simulink model "furuta_rl_training"  (R2026b)
settings: Solver=FixedStepDiscrete  StopTime=5  FixedStep=controlPeriod
model workspace (MAT data in the model file):
  agentKind = "PPO (초기 정책)"
  controlPeriod = 0.01
  controllerMode = 1
  furutaAgent : rl.agent.rlPPOAgent (value not decoded)
  furutaToolboxMpc = mpc
  furutaToolboxMpc.Ts = 0.01
  furutaToolboxMpc.PredictionHorizon = 20
  furutaToolboxMpc.ControlHorizon = 20
  furutaToolboxMpc.Model.Plant = ss
  furutaToolboxMpc.Model.Plant.InputName_ = "MV1"
  furutaToolboxMpc.Model.Plant.InputGroup_.Manipulated = 1
  furutaToolboxMpc.Model.Plant.OutputName_ = ["MO1"; "MO2"; "MO3"; "MO4"; "MO5"; "MO6"; "MO7"; "MO8"]
  furutaToolboxMpc.Model.Plant.OutputGroup_.Measured = [1 2 3 4 5 6 7 8]
  furutaToolboxMpc.Model.Plant.IOSize_ = [8 1]
  furutaToolboxMpc.Model.Plant.Data_ = ltipack.ssdata
  furutaToolboxMpc.Model.Plant.Data_.a = [1  -0.00902674267589  0.00993774320897  -2.4767657698e-05; 0  1.0129802947  5.33054368483e-05  0.0100355972733; 0  -1.80504476453  0.987560350231  -0.00796081332398; 0  2.59780112786  0.0106592935191  1.01144622057]
  furutaToolboxMpc.Model.Plant.Data_.c = [1  0  0  0; 0  1  0  0; 0  0  1  0; 0  0  0  1; 23.187012799  50.483540443  3.96076595787  4.74600329341; 0  69.1342012244  4.52520194197  5.64653884547; 0  0  1.92549619263  1.610475723; 0  0  0  1.43133536407]
  furutaToolboxMpc.Model.Plant.Data_.dx0 = [0; 0; 0; 0]
  furutaToolboxMpc.Model.Plant.Data_.x0 = [0; 0; 0; 0]
  furutaToolboxMpc.Model.Plant.Data_.b = [0.0186770373086; -0.0159916310545; 3.73189493068; -3.19778805573]
  furutaToolboxMpc.Model.Plant.Data_.d = [0; 0; 0; 0; 0; 0; 0; 0]
  furutaToolboxMpc.Model.Plant.Data_.u0 = 0
  furutaToolboxMpc.Model.Plant.Data_.y0 = [0; 0; 0; 0; 0; 0; 0; 0]
  furutaToolboxMpc.Model.Plant.Data_.Delay.Input = 0
  furutaToolboxMpc.Model.Plant.Data_.Delay.Output = [0; 0; 0; 0; 0; 0; 0; 0]
  furutaToolboxMpc.Model.Plant.Data_.Delay.Internal = []
  furutaToolboxMpc.Model.Plant.Data_.Ts = 0.01
  furutaToolboxMpc.Model.Disturbance = []
  furutaToolboxMpc.Model.Noise = []
  furutaToolboxMpc.Model.Nominal.X = [0; 0; 0; 0]
  furutaToolboxMpc.Model.Nominal.DX = [0; 0; 0; 0]
  furutaToolboxMpc.Model.Nominal.U = 0
  furutaToolboxMpc.Model.Nominal.Y = [0; 0; 0; 0; 0; 0; 0; 0]
  furutaToolboxMpc.ManipulatedVariables.Min = [-1; -1; -1; -1; -1; -1; -1; -1; -1; -1; -1; -1; -1; -1; -1; -1; -1; -1; -1; -1]
  furutaToolboxMpc.ManipulatedVariables.Max = [1; 1; 1; 1; 1; 1; 1; 1; 1; 1; 1; 1; 1; 1; 1; 1; 1; 1; 1; 1]
  furutaToolboxMpc.ManipulatedVariables.MinECR = [0; 0; 0; 0; 0; 0; 0; 0; 0; 0; 0; 0; 0; 0; 0; 0; 0; 0; 0; 0]
  furutaToolboxMpc.ManipulatedVariables.MaxECR = [0; 0; 0; 0; 0; 0; 0; 0; 0; 0; 0; 0; 0; 0; 0; 0; 0; 0; 0; 0]
  furutaToolboxMpc.ManipulatedVariables.RateMin = -Inf
  furutaToolboxMpc.ManipulatedVariables.RateMax = Inf
  furutaToolboxMpc.ManipulatedVariables.RateMinECR = 0
  furutaToolboxMpc.ManipulatedVariables.RateMaxECR = 0
  furutaToolboxMpc.ManipulatedVariables.Target = 'nominal'
  furutaToolboxMpc.ManipulatedVariables.Name = 'MV1'
  furutaToolboxMpc.ManipulatedVariables.Units = ''
  furutaToolboxMpc.ManipulatedVariables.ScaleFactor = 1
  furutaToolboxMpc.ManipulatedVariables.Type = 'continuous'
  furutaToolboxMpc.OutputVariables(1).Min = [-Inf; -Inf; -Inf; -Inf; -Inf; -Inf; -Inf; -Inf; -Inf; -Inf; -Inf; -Inf; -Inf; -Inf; -Inf; -Inf; -Inf; -Inf; -Inf; -Inf]
  furutaToolboxMpc.OutputVariables(1).Max = [Inf; Inf; Inf; Inf; Inf; Inf; Inf; Inf; Inf; Inf; Inf; Inf; Inf; Inf; Inf; Inf; Inf; Inf; Inf; Inf]
  furutaToolboxMpc.OutputVariables(1).MinECR = [2; 2; 2; 2; 2; 2; 2; 2; 2; 2; 2; 2; 2; 2; 2; 2; 2; 2; 2; 2]
  furutaToolboxMpc.OutputVariables(1).MaxECR = [2; 2; 2; 2; 2; 2; 2; 2; 2; 2; 2; 2; 2; 2; 2; 2; 2; 2; 2; 2]
  furutaToolboxMpc.OutputVariables(1).Name = 'MO1'
  furutaToolboxMpc.OutputVariables(1).Units = ''
  furutaToolboxMpc.OutputVariables(1).ScaleFactor = 1
  furutaToolboxMpc.OutputVariables(2).Min = [-Inf; -Inf; -Inf; -Inf; -Inf; -Inf; -Inf; -Inf; -Inf; -Inf; -Inf; -Inf; -Inf; -Inf; -Inf; -Inf; -Inf; -Inf; -Inf; -Inf]
  furutaToolboxMpc.OutputVariables(2).Max = [Inf; Inf; Inf; Inf; Inf; Inf; Inf; Inf; Inf; Inf; Inf; Inf; Inf; Inf; Inf; Inf; Inf; Inf; Inf; Inf]
  furutaToolboxMpc.OutputVariables(2).MinECR = [2; 2; 2; 2; 2; 2; 2; 2; 2; 2; 2; 2; 2; 2; 2; 2; 2; 2; 2; 2]
  furutaToolboxMpc.OutputVariables(2).MaxECR = [2; 2; 2; 2; 2; 2; 2; 2; 2; 2; 2; 2; 2; 2; 2; 2; 2; 2; 2; 2]
  furutaToolboxMpc.OutputVariables(2).Name = 'MO2'
  furutaToolboxMpc.OutputVariables(2).Units = ''
  furutaToolboxMpc.OutputVariables(2).ScaleFactor = 1
  furutaToolboxMpc.OutputVariables(3).Min = [-Inf; -Inf; -Inf; -Inf; -Inf; -Inf; -Inf; -Inf; -Inf; -Inf; -Inf; -Inf; -Inf; -Inf; -Inf; -Inf; -Inf; -Inf; -Inf; -Inf]
  furutaToolboxMpc.OutputVariables(3).Max = [Inf; Inf; Inf; Inf; Inf; Inf; Inf; Inf; Inf; Inf; Inf; Inf; Inf; Inf; Inf; Inf; Inf; Inf; Inf; Inf]
  furutaToolboxMpc.OutputVariables(3).MinECR = [2; 2; 2; 2; 2; 2; 2; 2; 2; 2; 2; 2; 2; 2; 2; 2; 2; 2; 2; 2]
  furutaToolboxMpc.OutputVariables(3).MaxECR = [2; 2; 2; 2; 2; 2; 2; 2; 2; 2; 2; 2; 2; 2; 2; 2; 2; 2; 2; 2]
  furutaToolboxMpc.OutputVariables(3).Name = 'MO3'
  furutaToolboxMpc.OutputVariables(3).Units = ''
  furutaToolboxMpc.OutputVariables(3).ScaleFactor = 1
  furutaToolboxMpc.OutputVariables(4).Min = [-Inf; -Inf; -Inf; -Inf; -Inf; -Inf; -Inf; -Inf; -Inf; -Inf; -Inf; -Inf; -Inf; -Inf; -Inf; -Inf; -Inf; -Inf; -Inf; -Inf]
  furutaToolboxMpc.OutputVariables(4).Max = [Inf; Inf; Inf; Inf; Inf; Inf; Inf; Inf; Inf; Inf; Inf; Inf; Inf; Inf; Inf; Inf; Inf; Inf; Inf; Inf]
  furutaToolboxMpc.OutputVariables(4).MinECR = [2; 2; 2; 2; 2; 2; 2; 2; 2; 2; 2; 2; 2; 2; 2; 2; 2; 2; 2; 2]
  furutaToolboxMpc.OutputVariables(4).MaxECR = [2; 2; 2; 2; 2; 2; 2; 2; 2; 2; 2; 2; 2; 2; 2; 2; 2; 2; 2; 2]
  furutaToolboxMpc.OutputVariables(4).Name = 'MO4'
  furutaToolboxMpc.OutputVariables(4).Units = ''
  furutaToolboxMpc.OutputVariables(4).ScaleFactor = 1
  furutaToolboxMpc.OutputVariables(5).Min = [-Inf; -Inf; -Inf; -Inf; -Inf; -Inf; -Inf; -Inf; -Inf; -Inf; -Inf; -Inf; -Inf; -Inf; -Inf; -Inf; -Inf; -Inf; -Inf; -Inf]
  furutaToolboxMpc.OutputVariables(5).Max = [Inf; Inf; Inf; Inf; Inf; Inf; Inf; Inf; Inf; Inf; Inf; Inf; Inf; Inf; Inf; Inf; Inf; Inf; Inf; Inf]
  furutaToolboxMpc.OutputVariables(5).MinECR = [2; 2; 2; 2; 2; 2; 2; 2; 2; 2; 2; 2; 2; 2; 2; 2; 2; 2; 2; 2]
  furutaToolboxMpc.OutputVariables(5).MaxECR = [2; 2; 2; 2; 2; 2; 2; 2; 2; 2; 2; 2; 2; 2; 2; 2; 2; 2; 2; 2]
  furutaToolboxMpc.OutputVariables(5).Name = 'MO5'
  furutaToolboxMpc.OutputVariables(5).Units = ''
  furutaToolboxMpc.OutputVariables(5).ScaleFactor = 1
  furutaToolboxMpc.OutputVariables(6).Min = [-Inf; -Inf; -Inf; -Inf; -Inf; -Inf; -Inf; -Inf; -Inf; -Inf; -Inf; -Inf; -Inf; -Inf; -Inf; -Inf; -Inf; -Inf; -Inf; -Inf]
  furutaToolboxMpc.OutputVariables(6).Max = [Inf; Inf; Inf; Inf; Inf; Inf; Inf; Inf; Inf; Inf; Inf; Inf; Inf; Inf; Inf; Inf; Inf; Inf; Inf; Inf]
  furutaToolboxMpc.OutputVariables(6).MinECR = [2; 2; 2; 2; 2; 2; 2; 2; 2; 2; 2; 2; 2; 2; 2; 2; 2; 2; 2; 2]
  furutaToolboxMpc.OutputVariables(6).MaxECR = [2; 2; 2; 2; 2; 2; 2; 2; 2; 2; 2; 2; 2; 2; 2; 2; 2; 2; 2; 2]
  furutaToolboxMpc.OutputVariables(6).Name = 'MO6'
  furutaToolboxMpc.OutputVariables(6).Units = ''
  furutaToolboxMpc.OutputVariables(6).ScaleFactor = 1
  furutaToolboxMpc.OutputVariables(7).Min = [-Inf; -Inf; -Inf; -Inf; -Inf; -Inf; -Inf; -Inf; -Inf; -Inf; -Inf; -Inf; -Inf; -Inf; -Inf; -Inf; -Inf; -Inf; -Inf; -Inf]
  furutaToolboxMpc.OutputVariables(7).Max = [Inf; Inf; Inf; Inf; Inf; Inf; Inf; Inf; Inf; Inf; Inf; Inf; Inf; Inf; Inf; Inf; Inf; Inf; Inf; Inf]
  furutaToolboxMpc.OutputVariables(7).MinECR = [2; 2; 2; 2; 2; 2; 2; 2; 2; 2; 2; 2; 2; 2; 2; 2; 2; 2; 2; 2]
  furutaToolboxMpc.OutputVariables(7).MaxECR = [2; 2; 2; 2; 2; 2; 2; 2; 2; 2; 2; 2; 2; 2; 2; 2; 2; 2; 2; 2]
  furutaToolboxMpc.OutputVariables(7).Name = 'MO7'
  furutaToolboxMpc.OutputVariables(7).Units = ''
  furutaToolboxMpc.OutputVariables(7).ScaleFactor = 1
  furutaToolboxMpc.OutputVariables(8).Min = [-Inf; -Inf; -Inf; -Inf; -Inf; -Inf; -Inf; -Inf; -Inf; -Inf; -Inf; -Inf; -Inf; -Inf; -Inf; -Inf; -Inf; -Inf; -Inf; -Inf]
  furutaToolboxMpc.OutputVariables(8).Max = [Inf; Inf; Inf; Inf; Inf; Inf; Inf; Inf; Inf; Inf; Inf; Inf; Inf; Inf; Inf; Inf; Inf; Inf; Inf; Inf]
  furutaToolboxMpc.OutputVariables(8).MinECR = [2; 2; 2; 2; 2; 2; 2; 2; 2; 2; 2; 2; 2; 2; 2; 2; 2; 2; 2; 2]
  furutaToolboxMpc.OutputVariables(8).MaxECR = [2; 2; 2; 2; 2; 2; 2; 2; 2; 2; 2; 2; 2; 2; 2; 2; 2; 2; 2; 2]
  furutaToolboxMpc.OutputVariables(8).Name = 'MO8'
  furutaToolboxMpc.OutputVariables(8).Units = ''
  furutaToolboxMpc.OutputVariables(8).ScaleFactor = 1
  furutaToolboxMpc.Weights.ManipulatedVariables = [1; 1; 1; 1; 1; 1; 1; 1; 1; 1; 1; 1; 1; 1; 1; 1; 1; 1; 1; 1]
  furutaToolboxMpc.Weights.ManipulatedVariablesRate = 1e-05
  furutaToolboxMpc.Weights.OutputVariables = [3.16227766017  3.16227766017  1  1  0  0  0  0; 3.16227766017  3.16227766017  1  1  0  0  0  0; 3.16227766017  3.16227766017  1  1  0  0  0  0; 3.16227766017  3.16227766017  1  1  0  0  0  0; 3.16227766017  3.16227766017  1  1  0  0  0  0; 3.16227766017  3.16227766017  1  1  0  0  0  0; 3.16227766017  3.16227766017  1  1  0  0  0  0; 3.16227766017  3.16227766017  1  1  0  0  0  0; 3.16227766017  3.16227766017  1  1  0  0  0  0; 3.16227766017  3.16227766017  1  1  0  0  0  0; 3.16227766017  3.16227766017  1  1  0  0  0  0; 3.16227766017  3.16227766017  1  1  0  0  0  0; 3.16227766017  3.16227766017  1  1  0  0  0  0; 3.16227766017  3.16227766017  1  1  0  0  0  0; 3.16227766017  3.16227766017  1  1  0  0  0  0; 3.16227766017  3.16227766017  1  1  0  0  0  0; 3.16227766017  3.16227766017  1  1  0  0  0  0; 3.16227766017  3.16227766017  1  1  0  0  0  0; 3.16227766017  3.16227766017  1  1  0  0  0  0; 0  0  0  0  1  1  1  1]
  furutaToolboxMpc.Weights.ECR = 100000
  furutaToolboxMpc.Optimizer.OptimizationType = 'QP'
  furutaToolboxMpc.Optimizer.Solver = 'active-set'
  furutaToolboxMpc.Optimizer.SolverOptions = mpc.solver.options.qp.ActiveSet
  furutaToolboxMpc.Optimizer.SolverOptions.SolverName = 'ActiveSet'
  furutaToolboxMpc.Optimizer.MinOutputECR = 0
  furutaToolboxMpc.Optimizer.UseSuboptimalSolution = 0
  furutaToolboxMpc.Optimizer.CustomSolver = 0
  furutaToolboxMpc.Optimizer.CustomSolverCodeGen = 0
  furutaToolboxMpc.History = [2026 11 18 15 19 42.726]
  furutaToolboxMpc.MPCData = mpcdata
  furutaToolboxMpc.MPCData.IsDirty = 1
  furutaToolboxMpc.MPCData.Ts = 0.01
  furutaToolboxMpc.MPCData.p = 20
  furutaToolboxMpc.MPCData.m = 20
  furutaToolboxMpc.MPCData.UseActiveSetSolver = 1
  furutaToolboxMpc.MPCData.UseSuboptimalSolution = 0
  furutaToolboxMpc.MPCData.CustomSolver = 0
  furutaToolboxMpc.MPCData.CustomSolverCodeGen = 0
  furutaToolboxMpc.MPCData.IsCustomEstimation = 1
  furutaToolboxMpc.MPCData.Uscale = 1
  furutaToolboxMpc.MPCData.Yscale = [1; 1; 1; 1; 1; 1; 1; 1]
  furutaToolboxMpc.MPCData.mvindex = 1
  furutaToolboxMpc.MPCData.myindex = [1; 2; 3; 4; 5; 6; 7; 8]
  furutaToolboxMpc.MPCData.ASOptions.MaxIterations = 120
  furutaToolboxMpc.MPCData.ASOptions.MaxTime = Inf
  furutaToolboxMpc.MPCData.ASOptions.ConstraintTolerance = 1e-06
  furutaToolboxMpc.MPCData.ASOptions.UseWarmStart = 1
  furutaToolboxMpc.MPCData.IPOptions.MaxIterations = 50
  furutaToolboxMpc.MPCData.IPOptions.MaxTime = Inf
  furutaToolboxMpc.MPCData.IPOptions.ConstraintTolerance = 1e-06
  furutaToolboxMpc.MPCData.IPOptions.OptimalityTolerance = 1e-06
  furutaToolboxMpc.MPCData.IPOptions.ComplementarityTolerance = 1e-08
  furutaToolboxMpc.MPCData.IPOptions.StepTolerance = 1e-08
  furutaToolboxMpc.MPCData.ADOptions.AbsoluteTolerance = 0.001
  furutaToolboxMpc.MPCData.ADOptions.RelativeTolerance = 0.001
  furutaToolboxMpc.MPCData.ADOptions.MaxIterations = 1000
  furutaToolboxMpc.MPCData.ADOptions.MaxTime = Inf
  furutaToolboxMpc.MPCData.ADOptions.RelaxationParameter = 1.6
  furutaToolboxMpc.MPCData.ADOptions.PenaltyParameter = 0.1
  furutaToolboxMpc.MPCData.ADOptions.StepSize = 1e-06
  furutaToolboxMpc.MPCData.ADOptions.PrimalInfeasibilityTolerance = 0.0001
  furutaToolboxMpc.MPCData.ADOptions.DualInfeasibilityTolerance = 0.0001
  furutaToolboxMpc.MPCData.ADOptions.EnablePolish = 0
  furutaToolboxMpc.MPCData.ADOptions.PolishRegularization = 1e-06
  furutaToolboxMpc.MPCData.ADOptions.PolishTolerance = 1e-08
  furutaToolboxMpc.MPCData.ADOptions.PolishMaxIterations = 3
  furutaToolboxMpc.MPCData.MIQPOptions.MaxIterations = 1000
  furutaToolboxMpc.MPCData.MIQPOptions.MaxTime = Inf
  furutaToolboxMpc.MPCData.MIQPOptions.ConstraintTolerance = 1e-06
  furutaToolboxMpc.MPCData.MIQPOptions.UseWarmStart = 0
  furutaToolboxMpc.MPCData.MIQPOptions.DiscreteConstraintTolerance = 1e-06
  furutaToolboxMpc.MPCData.MIQPOptions.RoundingAtRootNode = 1
  furutaToolboxMpc.MPCData.MIQPOptions.MaxPendingNodes = 1000
  furutaToolboxMpc.IsEmpty = 0
  furutaToolboxMpc.OldOVIntegrator = {[]; []; []; []; []; []; []; []}
  furutaToolboxMpc.EstGain = 'custom'
  furutaToolboxMpc.OutDistModel = ss
  furutaToolboxMpc.OutDistModel.IOSize_ = [8 1]
  furutaToolboxMpc.OutDistModel.Data_ = ltipack.ssdata
  furutaToolboxMpc.OutDistModel.Data_.d = [0; 0; 0; 0; 0; 0; 0; 0]
  furutaToolboxMpc.OutDistModel.Data_.u0 = 0
  furutaToolboxMpc.OutDistModel.Data_.y0 = [0; 0; 0; 0; 0; 0; 0; 0]
  furutaToolboxMpc.OutDistModel.Data_.Delay.Input = 0
  furutaToolboxMpc.OutDistModel.Data_.Delay.Output = [0; 0; 0; 0; 0; 0; 0; 0]
  furutaToolboxMpc.OutDistModel.Data_.Delay.Internal = []
  furutaToolboxMpc.OutDistModel.Data_.Ts = 0
  furutaToolboxMpc.Version = '26.2'
  initialState = [0; 0.174532925199; 0; 0]
  integrationStep = 0.002
  lmpcF = [-2830.68997815  -425545.566766  -3378.75183897  -27996.6485902; -2386.43056313  -361642.554145  -2861.88762577  -23784.8995788; -2007.92623528  -307039.935727  -2420.70891761  -20186.6799153; -1685.61022299  -260385.70884  -2044.21747245  -17112.76233; -1411.30389107  -220523.512325  -1723.00852583  -14486.8389364; -1178.01505811  -186464.084025  -1449.03879544  -12243.6357575; -979.765570681  -157360.828718  -1215.42801756  -10327.2990171; -811.443882151  -132488.892998  -1016.2891174  -8690.01329063; -668.67900017  -111227.229747  -846.5828196  -7290.81731336; -547.732694122  -93043.2082769  -701.993107015  -6094.58810591; -445.407303829  -77479.3885256  -578.820447971  -5071.16820406; -358.966875555  -64142.130684  -473.890148738  -4194.61428813; -286.069679883  -52691.7563221  -384.473558738  -3442.54847023; -224.710446621  -42834.0147656  -308.220170492  -2795.59599508; -173.170891379  -34312.6399545  -243.098922081  -2236.8951992; -129.97731279  -26902.8090841  -187.34723347  -1751.66730548; -93.8642135106  -20405.3356068  -139.426494783  -1326.83504718; -63.7430465086  -14641.4461488  -97.9828790679  -950.680248883; -38.6753142339  -9448.00396528  -61.8124779305  -612.531370742; -17.8493553576  -4673.05100156  -29.8298585475  -302.472662498]
  lmpcH = [71196.7632757 60515.4631775 51389.63963 43592.1776843 36929.7000861 31236.7872342 26371.8858267 22213.8049684 18658.7129743 15617.560407 13013.8653496 10781.8057824 ... (400 elements, 20x20)]
  lqrGain = [-0.560244322113 -7.30813603654 -0.304541725168 -0.68699829167]
  maxTorque = 0.03
  pidGains = [8.3479 0.5085 0.5811 0.3312 0.0475]
  plantCoefficients = [0.00019818 0.00016078 0.00016134 0.00013805 0.016934 0.0001 1e-05 0]
  poleGain = [-1.34079378819 -10.2715412157 -0.553426126336 -0.956316780761]
  rlRewardLevel = 2
  rmd.model = 'RMD-X6-P20-60-E'
  rmd.voltage = 48
  rmd.gearRatio = 19.612
  rmd.ratedTorque = 20
  rmd.ratedCurrent = 9.5
  rmd.ratedSpeedRPM = 153
  rmd.noLoadSpeedRPM = 176
  rmd.Kt = 2.1
  rmd.currentLSB = 0.01
  rmdCommandDelaySamples = 1
  rmdCurrentTimeConstant = 0
  scenarioStimulus = [0 0.0075 0.0175 0.0275 0.0375 0.0475 0.0575 0.0675 0.0775 0.0875 0.0975 0.1075 ... (2004 elements, 501x4)]
  usePolicyCallback = 0
  useRmd = 1
undefined symbols (not defined in the file or in its folder): sgn
libraries: mpclib x1, rllib x1
(part 1 of 2)
settings Model: Creator=Lsh  LastModifiedBy=Lsh

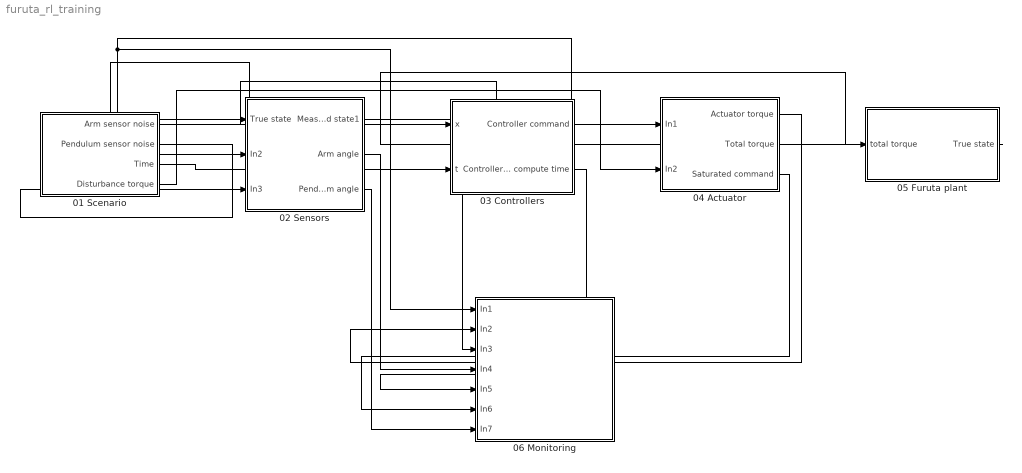
== system furuta_rl_training ==
  01 Scenario : Subsystem
  02 Sensors : Subsystem
  03 Controllers : Subsystem
  04 Actuator : Subsystem
  05 Furuta plant : Subsystem
  06 Monitoring : Subsystem
  wires:
  01 Scenario/1(Arm sensor noise) -> 02 Sensors/2(In2)
  01 Scenario/2(Pendulum sensor noise) -> 02 Sensors/3(In3)
  03 Controllers/1(Controller command) -> 06 Monitoring/3(In3), 04 Actuator/1(In1)
  02 Sensors/1(Measured state1) -> 03 Controllers/1(x)
  01 Scenario/3(Time) -> 03 Controllers/2(t)
  01 Scenario/4(Disturbance torque) -> 04 Actuator/2(In2)
  05 Furuta plant/1(True state) -> 06 Monitoring/1(In1), 02 Sensors/1(True state)
  04 Actuator/2(Total torque) -> 05 Furuta plant/1(total torque)
  04 Actuator/1(Actuator torque) -> 06 Monitoring/2(In2)
  02 Sensors/2(Arm angle) -> 06 Monitoring/4(In4)
  03 Controllers/2(Controller compute time) -> 06 Monitoring/5(In5)
  04 Actuator/3(Saturated command) -> 06 Monitoring/6(In6)
  02 Sensors/3(Pendulum angle) -> 06 Monitoring/7(In7)

== system furuta_rl_training/01 Scenario ==
  Clock : DigitalClock  SampleTime=controlPeriod
  Scenario : FromWorkspace  VariableName=scenarioStimulus  SampleTime=controlPeriod  Interpolate=off  OutputAfterFinalValue=Holding final value
  Scenario channels : Demux  Outputs=3
  Arm sensor noise : Outport
  Pendulum sensor noise : Outport  Port=2
  Time : Outport  Port=3
  Disturbance torque : Outport  Port=4
  wires:
  Scenario channels/1 -> Arm sensor noise/1  "Arm sensor noise"
  Clock/1 -> Time/1  "Time"
  Scenario/1 -> Scenario channels/1
  Scenario channels/3 -> Disturbance torque/1  "Disturbance torque"
  Scenario channels/2 -> Pendulum sensor noise/1  "Pendulum sensor noise"

== system furuta_rl_training/02 Sensors ==
  True state : Inport
  In2 : Inport  Port=2
  In3 : Inport  Port=3
  Measured arm : Sum
  Measured pendulum : Sum
  Measured state : Mux
  State channels : Demux
  Measured state1 : Outport
  Arm angle : Outport  Port=2
  Pendulum angle : Outport  Port=3
  wires:
  True state/1 -> State channels/1
  State channels/1 -> Arm angle/1, Measured arm/1  "Arm angle"
  Measured state/1 -> Measured state1/1  "Measured state"
  State channels/2 -> Pendulum angle/1, Measured pendulum/1  "Pendulum angle"
  Measured arm/1 -> Measured state/1
  Measured pendulum/1 -> Measured state/2
  State channels/4 -> Measured state/4
  State channels/3 -> Measured state/3
  In2/1 -> Measured arm/2
  In3/1 -> Measured pendulum/2

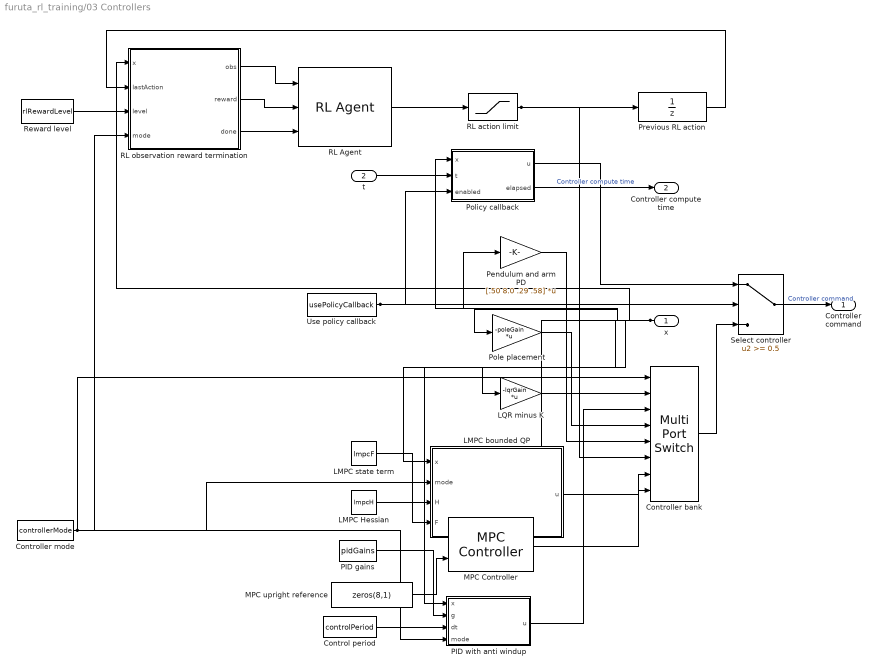
== system furuta_rl_training/03 Controllers ==
  x : Inport
  t : Inport  Port=2
  Control period : Constant  Value=controlPeriod
  Controller bank : MultiPortSwitch  Inputs=7  SaturateOnIntegerOverflow=off  InputSameDT=off
  Controller mode : Constant  Value=controllerMode
  LMPC Hessian : Constant  Value=lmpcH
  LMPC bounded QP : MATLAB Function  TreatAsAtomicUnit=on
  LMPC state term : Constant  Value=lmpcF
  LQR minus K : Gain  Gain=-lqrGain  Multiplication=Matrix(K*u) (u vector)
  MPC Controller : mpclib/MPC Controller  SCDEnableBlockLinearizationSpecification=on  mpcobj=furutaToolboxMpc  is_multiple=0  enable_value=0  return_u0=off  updateMPCinCallerWorkspace=on  md_inport=off  mv_inport=off  uref_inport=off  return_cost=off  return_mvseq=off  return_qpstatus=off  return_xseq=off  return_state=off  return_ovseq=off  state_inport=on  umin_inport=off  umax_inport=off  ymin_inport=off  ymax_inport=off  cc_inport=off  ywt_inport=off  uwt_inport=off  duwt_inport=off  rhoeps_inport=off  pm_inport=off  MaximumP=10  HorizonChoice=FixedHorizon  n_ts=1  n_p=10  n_mv=1  n_md=1  n_ud=0  n_mo=1  n_uo=0  BlockDataType=double  SampleTimeInherited=off  switch_inport=off
  MPC upright reference : Constant  Value=zeros(8,1)
  PID gains : Constant  Value=pidGains
  PID with anti windup : MATLAB Function  TreatAsAtomicUnit=on
  Pendulum and arm PD : Gain  Gain=[.50 8.0 .29 .58]  Multiplication=Matrix(K*u) (u vector)
  Pole placement : Gain  Gain=-poleGain  Multiplication=Matrix(K*u) (u vector)
  Policy callback : MATLAB Function  TreatAsAtomicUnit=on
  Previous RL action : UnitDelay  SampleTime=controlPeriod
  RL Agent : rllib/RL Agent  Agent=furutaAgent  ExternalActionAsInput=off  ProvideLastAction=off  ProvideCumRwd=off  TreatAsDirectFeedthrough=on  UseStrictObservationDataTypes=off
  RL action limit : Saturate  UpperLimit=1  LowerLimit=-1
  RL observation reward termination : MATLAB Function  TreatAsAtomicUnit=on
  Reward level : Constant  Value=rlRewardLevel
  Select controller : Switch  Threshold=0.5  SaturateOnIntegerOverflow=off  InputSameDT=off
  Use policy callback : Constant  Value=usePolicyCallback
  Controller command : Outport
  Controller compute time : Outport  Port=2
  wires:
  Reward level/1 -> RL observation reward termination/3(level)
  RL observation reward termination/2(reward) -> RL Agent/2
  Controller mode/1 -> PID with anti windup/4(mode), LMPC bounded QP/2(mode), Controller bank/1, RL observation reward termination/4(mode)
  LMPC Hessian/1 -> LMPC bounded QP/3(H)
  Use policy callback/1 -> Select controller/2, Policy callback/3(enabled)
  RL observation reward termination/1(obs) -> RL Agent/1
  RL observation reward termination/3(done) -> RL Agent/3
  RL Agent/1 -> RL action limit/1
  t/1 -> Policy callback/2(t)
  LMPC state term/1 -> LMPC bounded QP/4(F)
  PID gains/1 -> PID with anti windup/2(g)
  Control period/1 -> PID with anti windup/3(dt)
  RL action limit/1 -> Previous RL action/1, Controller bank/6
  Policy callback/1(u) -> Select controller/1
  Policy callback/2(elapsed) -> Controller compute time/1  "Controller compute time"
  Pendulum and arm PD/1 -> Controller bank/5
  Pole placement/1 -> Controller bank/4
  LQR minus K/1 -> Controller bank/2
  LMPC bounded QP/1(u) -> Controller bank/7
  Select controller/1 -> Controller command/1  "Controller command"
  PID with anti windup/1(u) -> Controller bank/3
  x/1 -> Pole placement/1, LQR minus K/1, LMPC bounded QP/1(x), Policy callback/1(x), Pendulum and arm PD/1, PID with anti windup/1(x), RL observation reward termination/1(x), MPC Controller/1
  Previous RL action/1 -> RL observation reward termination/2(lastAction)
  Controller bank/1 -> Select controller/3
  MPC upright reference/1 -> MPC Controller/2
  MPC Controller/1 -> Controller bank/8

== system furuta_rl_training/04 Actuator ==
  In1 : Inport
  In2 : Inport  Port=2
  Actuator limits : Saturate  UpperLimit=1  LowerLimit=-1
  Add disturbance : Sum
  Applied torque log : ToWorkspace  VariableName=appliedTorqueTrace  SampleTime=-1
  RMD X6 P20 60 E : Subsystem
  Select actuator : Switch  Threshold=0.5  SaturateOnIntegerOverflow=off  InputSameDT=off
  Torque Nm : Gain  Gain=maxTorque
  Use RMD : Constant  Value=useRmd
  Actuator torque : Outport
  Total torque : Outport  Port=2
  Saturated command : Outport  Port=3
  wires:
  Use RMD/1 -> Select actuator/2
  In1/1 -> Actuator limits/1
  RMD X6 P20 60 E/1(Output torque) -> Select actuator/1
  Actuator limits/1 -> Saturated command/1, Torque Nm/1  "Saturated command"
  Select actuator/1 -> Actuator torque/1, Applied torque log/1, Add disturbance/1
  Torque Nm/1 -> Select actuator/3, RMD X6 P20 60 E/1(Requested torque)  "Actuator torque"
  In2/1 -> Add disturbance/2
  Add disturbance/1 -> Total torque/1  "Total torque"

== system furuta_rl_training/05 Furuta plant ==
  total torque : Inport
  Plant state : UnitDelay  InitialCondition=initialState  SampleTime=controlPeriod
  RK4 Furuta plant : Subsystem
  True state : Outport
  wires:
  RK4 Furuta plant/1(next state) -> Plant state/1
  Plant state/1 -> RK4 Furuta plant/1(state), True state/1  "True state"
  total torque/1 -> RK4 Furuta plant/2(total torque)

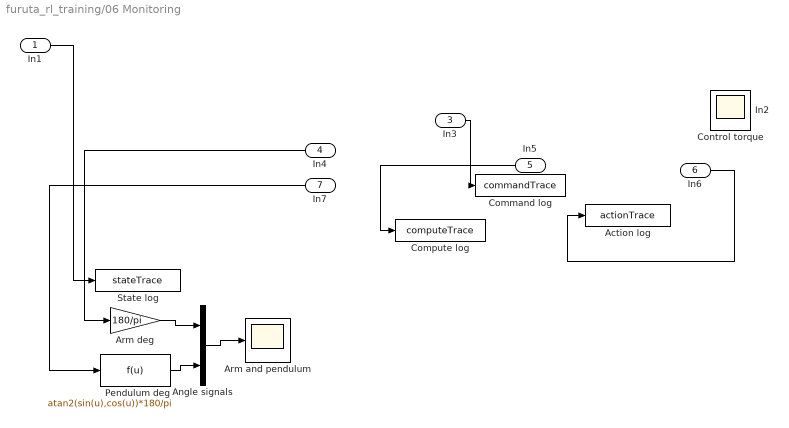
== system furuta_rl_training/06 Monitoring ==
  In1 : Inport
  In2 : Inport  Port=2
  In3 : Inport  Port=3
  In4 : Inport  Port=4
  In5 : Inport  Port=5
  In6 : Inport  Port=6
  In7 : Inport  Port=7
  Action log : ToWorkspace  VariableName=actionTrace  SampleTime=-1
  Angle signals : Mux  Inputs=2
  Arm and pendulum : Scope
  Arm deg : Gain  Gain=180/pi
  Command log : ToWorkspace  VariableName=commandTrace  SampleTime=-1
  Compute log : ToWorkspace  VariableName=computeTrace  SampleTime=-1
  Control torque : Scope
  Pendulum deg : Fcn  Expr=atan2(sin(u),cos(u))*180/pi
  State log : ToWorkspace  VariableName=stateTrace  SampleTime=-1
  wires:
  Pendulum deg/1 -> Angle signals/2
  In4/1 -> Arm deg/1
  Arm deg/1 -> Angle signals/1
  Angle signals/1 -> Arm and pendulum/1
  In3/1 -> Command log/1
  In1/1 -> State log/1
  In5/1 -> Compute log/1
  In2/1 -> Control torque/1
  In6/1 -> Action log/1
  In7/1 -> Pendulum deg/1

== system furuta_rl_training/04 Actuator/RMD X6 P20 60 E ==
  Requested torque : Inport
  Command delay : Delay  DelayLength=rmdCommandDelaySamples  SampleTime=controlPeriod
  Counts to current : Gain  Gain=rmd.currentLSB
  Current count limit : Saturate  UpperLimit=floor(min([maxTorque/rmd.Kt rmd.ratedTorque/rmd.Kt rmd.ratedCurrent])/rmd.currentLSB)  LowerLimit=-(floor(min([maxTorque/rmd.Kt rmd.ratedTorque/rmd.Kt rmd.ratedCurrent])/rmd.currentLSB))
  Current log : ToWorkspace  VariableName=rmdCurrentTrace  SampleTime=-1
  Current tracking : DiscreteTransferFcn  Numerator=[1-exp(-controlPeriod/max(rmdCurrentTimeConstant,eps)) 0]  Denominator=[1 -exp(-controlPeriod/max(rmdCurrentTimeConstant,eps))]  SampleTime=controlPeriod
  Output Kt : Gain  Gain=rmd.Kt
  Quantize A1 : Rounding  Operator=round
  Torque to A1 counts : Gain  Gain=1/(rmd.Kt*rmd.currentLSB)
  Output torque : Outport
  wires:
  Requested torque/1 -> Torque to A1 counts/1
  Torque to A1 counts/1 -> Quantize A1/1
  Quantize A1/1 -> Current count limit/1
  Current count limit/1 -> Command delay/1
  Command delay/1 -> Counts to current/1
  Counts to current/1 -> Current tracking/1
  Current tracking/1 -> Output Kt/1, Current log/1
  Output Kt/1 -> Output torque/1

== system furuta_rl_training/05 Furuta plant/RK4 Furuta plant ==
  state : Inport
  total torque : Inport  Port=2
  Substep 1 : Subsystem
  Substep 2 : Subsystem
  Substep 3 : Subsystem
  Substep 4 : Subsystem
  Substep 5 : Subsystem
  next state : Outport
  wires:
  state/1 -> Substep 1/1(x)
  total torque/1 -> Substep 1/2(tau), Substep 2/2(tau), Substep 3/2(tau), Substep 4/2(tau), Substep 5/2(tau)
  Substep 1/1(x next) -> Substep 2/1(x)
  Substep 2/1(x next) -> Substep 3/1(x)
  Substep 3/1(x next) -> Substep 4/1(x)
  Substep 4/1(x next) -> Substep 5/1(x)
  Substep 5/1(x next) -> next state/1

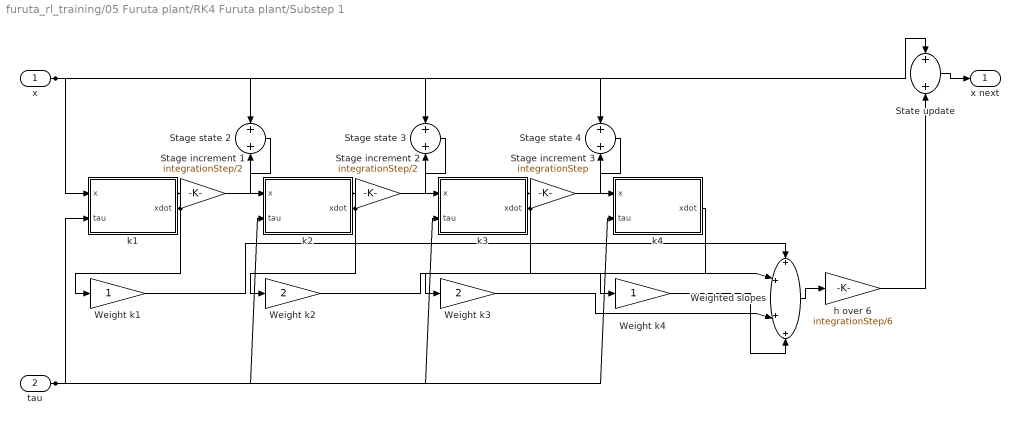
== system furuta_rl_training/05 Furuta plant/RK4 Furuta plant/Substep 1 ==
  x : Inport
  tau : Inport  Port=2
  Stage increment 1 : Gain  Gain=integrationStep/2
  Stage increment 2 : Gain  Gain=integrationStep/2
  Stage increment 3 : Gain  Gain=integrationStep
  Stage state 2 : Sum
  Stage state 3 : Sum
  Stage state 4 : Sum
  State update : Sum
  Weight k1 : Gain
  Weight k2 : Gain  Gain=2
  Weight k3 : Gain  Gain=2
  Weight k4 : Gain
  Weighted slopes : Sum  Inputs=++++
  h over 6 : Gain  Gain=integrationStep/6
  k1 : Subsystem
  k2 : Subsystem
  k3 : Subsystem
  k4 : Subsystem
  x next : Outport
  wires:
  x/1 -> k1/1(x), Stage state 2/1, Stage state 3/1, Stage state 4/1, State update/1
  tau/1 -> k1/2(tau), k2/2(tau), k3/2(tau), k4/2(tau)
  k1/1(xdot) -> Stage increment 1/1, Weight k1/1
  Stage increment 1/1 -> Stage state 2/2
  Stage state 2/1 -> k2/1(x)
  k2/1(xdot) -> Stage increment 2/1, Weight k2/1
  Stage increment 2/1 -> Stage state 3/2
  Stage state 3/1 -> k3/1(x)
  k3/1(xdot) -> Stage increment 3/1, Weight k3/1
  Stage increment 3/1 -> Stage state 4/2
  Stage state 4/1 -> k4/1(x)
  k4/1(xdot) -> Weight k4/1
  Weight k1/1 -> Weighted slopes/1
  Weight k2/1 -> Weighted slopes/2
  Weight k3/1 -> Weighted slopes/3
  Weight k4/1 -> Weighted slopes/4
  Weighted slopes/1 -> h over 6/1
  h over 6/1 -> State update/2
  State update/1 -> x next/1

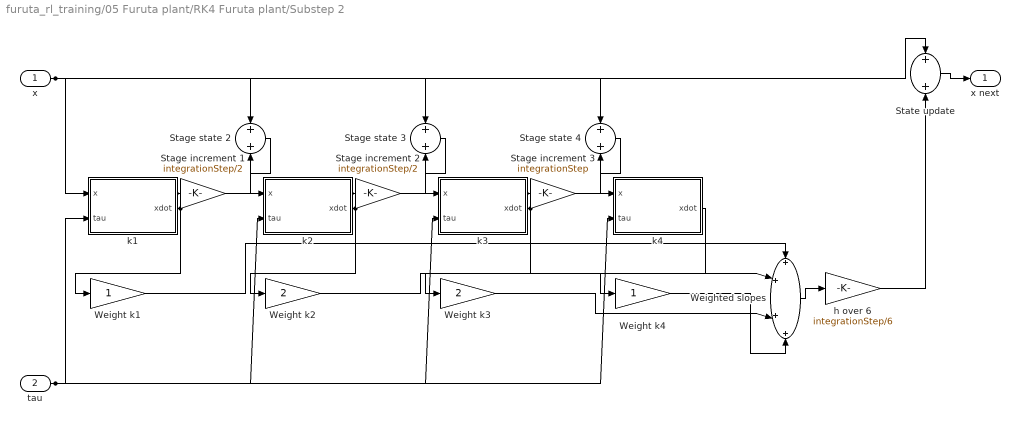
== system furuta_rl_training/05 Furuta plant/RK4 Furuta plant/Substep 2 ==
  x : Inport
  tau : Inport  Port=2
  Stage increment 1 : Gain  Gain=integrationStep/2
  Stage increment 2 : Gain  Gain=integrationStep/2
  Stage increment 3 : Gain  Gain=integrationStep
  Stage state 2 : Sum
  Stage state 3 : Sum
  Stage state 4 : Sum
  State update : Sum
  Weight k1 : Gain
  Weight k2 : Gain  Gain=2
  Weight k3 : Gain  Gain=2
  Weight k4 : Gain
  Weighted slopes : Sum  Inputs=++++
  h over 6 : Gain  Gain=integrationStep/6
  k1 : Subsystem
  k2 : Subsystem
  k3 : Subsystem
  k4 : Subsystem
  x next : Outport
  wires:
  State update/1 -> x next/1
  h over 6/1 -> State update/2
  Weighted slopes/1 -> h over 6/1
  Weight k4/1 -> Weighted slopes/4
  Weight k3/1 -> Weighted slopes/3
  Weight k2/1 -> Weighted slopes/2
  Weight k1/1 -> Weighted slopes/1
  k4/1(xdot) -> Weight k4/1
  Stage state 4/1 -> k4/1(x)
  Stage increment 3/1 -> Stage state 4/2
  k3/1(xdot) -> Weight k3/1, Stage increment 3/1
  Stage state 3/1 -> k3/1(x)
  Stage increment 2/1 -> Stage state 3/2
  k2/1(xdot) -> Weight k2/1, Stage increment 2/1
  Stage state 2/1 -> k2/1(x)
  Stage increment 1/1 -> Stage state 2/2
  k1/1(xdot) -> Weight k1/1, Stage increment 1/1
  tau/1 -> k4/2(tau), k3/2(tau), k2/2(tau), k1/2(tau)
  x/1 -> State update/1, Stage state 4/1, Stage state 3/1, Stage state 2/1, k1/1(x)

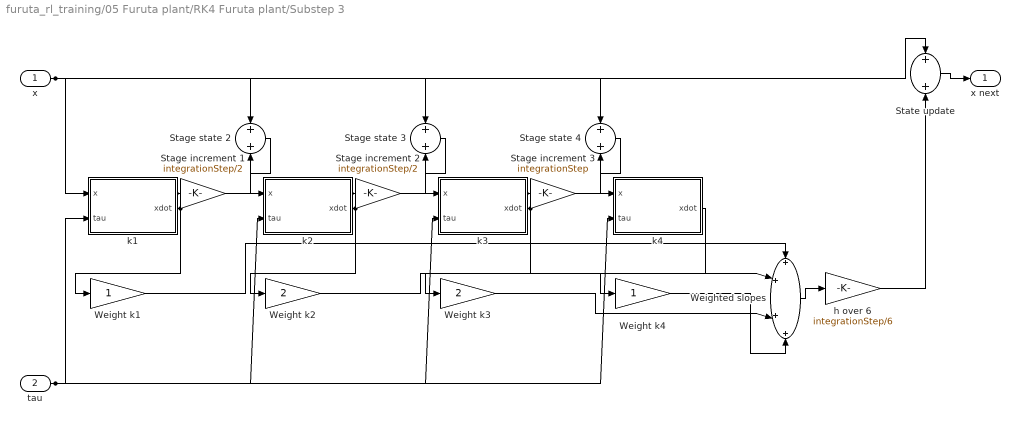
== system furuta_rl_training/05 Furuta plant/RK4 Furuta plant/Substep 3 ==
  x : Inport
  tau : Inport  Port=2
  Stage increment 1 : Gain  Gain=integrationStep/2
  Stage increment 2 : Gain  Gain=integrationStep/2
  Stage increment 3 : Gain  Gain=integrationStep
  Stage state 2 : Sum
  Stage state 3 : Sum
  Stage state 4 : Sum
  State update : Sum
  Weight k1 : Gain
  Weight k2 : Gain  Gain=2
  Weight k3 : Gain  Gain=2
  Weight k4 : Gain
  Weighted slopes : Sum  Inputs=++++
  h over 6 : Gain  Gain=integrationStep/6
  k1 : Subsystem
  k2 : Subsystem
  k3 : Subsystem
  k4 : Subsystem
  x next : Outport
  wires:
  State update/1 -> x next/1
  h over 6/1 -> State update/2
  Weighted slopes/1 -> h over 6/1
  Weight k4/1 -> Weighted slopes/4
  Weight k3/1 -> Weighted slopes/3
  Weight k2/1 -> Weighted slopes/2
  Weight k1/1 -> Weighted slopes/1
  k4/1(xdot) -> Weight k4/1
  Stage state 4/1 -> k4/1(x)
  Stage increment 3/1 -> Stage state 4/2
  k3/1(xdot) -> Weight k3/1, Stage increment 3/1
  Stage state 3/1 -> k3/1(x)
  Stage increment 2/1 -> Stage state 3/2
  k2/1(xdot) -> Weight k2/1, Stage increment 2/1
  Stage state 2/1 -> k2/1(x)
  Stage increment 1/1 -> Stage state 2/2
  k1/1(xdot) -> Weight k1/1, Stage increment 1/1
  tau/1 -> k4/2(tau), k3/2(tau), k2/2(tau), k1/2(tau)
  x/1 -> State update/1, Stage state 4/1, Stage state 3/1, Stage state 2/1, k1/1(x)

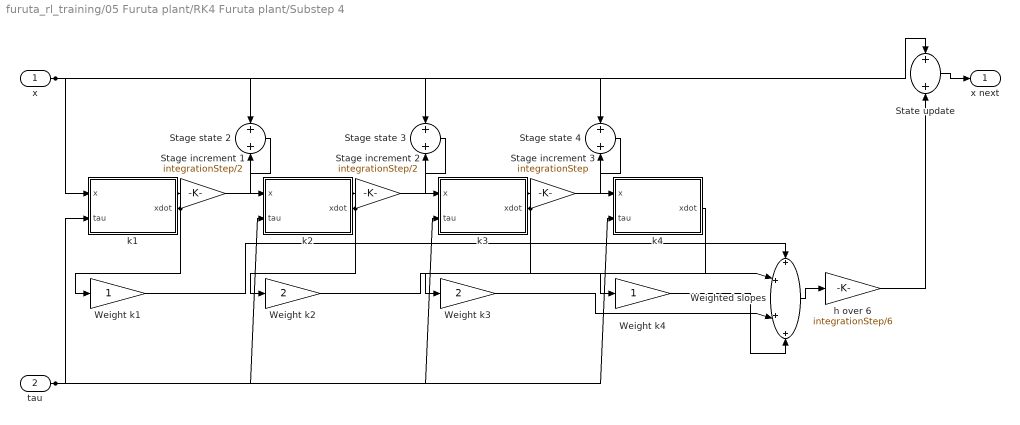
== system furuta_rl_training/05 Furuta plant/RK4 Furuta plant/Substep 4 ==
  x : Inport
  tau : Inport  Port=2
  Stage increment 1 : Gain  Gain=integrationStep/2
  Stage increment 2 : Gain  Gain=integrationStep/2
  Stage increment 3 : Gain  Gain=integrationStep
  Stage state 2 : Sum
  Stage state 3 : Sum
  Stage state 4 : Sum
  State update : Sum
  Weight k1 : Gain
  Weight k2 : Gain  Gain=2
  Weight k3 : Gain  Gain=2
  Weight k4 : Gain
  Weighted slopes : Sum  Inputs=++++
  h over 6 : Gain  Gain=integrationStep/6
  k1 : Subsystem
  k2 : Subsystem
  k3 : Subsystem
  k4 : Subsystem
  x next : Outport
  wires:
  State update/1 -> x next/1
  h over 6/1 -> State update/2
  Weighted slopes/1 -> h over 6/1
  Weight k4/1 -> Weighted slopes/4
  Weight k3/1 -> Weighted slopes/3
  Weight k2/1 -> Weighted slopes/2
  Weight k1/1 -> Weighted slopes/1
  k4/1(xdot) -> Weight k4/1
  Stage state 4/1 -> k4/1(x)
  Stage increment 3/1 -> Stage state 4/2
  k3/1(xdot) -> Weight k3/1, Stage increment 3/1
  Stage state 3/1 -> k3/1(x)
  Stage increment 2/1 -> Stage state 3/2
  k2/1(xdot) -> Weight k2/1, Stage increment 2/1
  Stage state 2/1 -> k2/1(x)
  Stage increment 1/1 -> Stage state 2/2
  k1/1(xdot) -> Weight k1/1, Stage increment 1/1
  tau/1 -> k4/2(tau), k3/2(tau), k2/2(tau), k1/2(tau)
  x/1 -> State update/1, Stage state 4/1, Stage state 3/1, Stage state 2/1, k1/1(x)

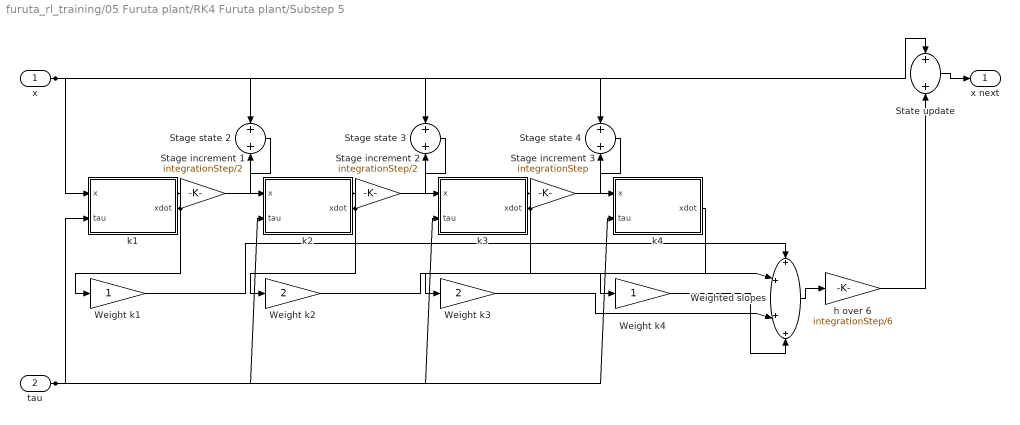
== system furuta_rl_training/05 Furuta plant/RK4 Furuta plant/Substep 5 ==
  x : Inport
  tau : Inport  Port=2
  Stage increment 1 : Gain  Gain=integrationStep/2
  Stage increment 2 : Gain  Gain=integrationStep/2
  Stage increment 3 : Gain  Gain=integrationStep
  Stage state 2 : Sum
  Stage state 3 : Sum
  Stage state 4 : Sum
  State update : Sum
  Weight k1 : Gain
  Weight k2 : Gain  Gain=2
  Weight k3 : Gain  Gain=2
  Weight k4 : Gain
  Weighted slopes : Sum  Inputs=++++
  h over 6 : Gain  Gain=integrationStep/6
  k1 : Subsystem
  k2 : Subsystem
  k3 : Subsystem
  k4 : Subsystem
  x next : Outport
  wires:
  State update/1 -> x next/1
  h over 6/1 -> State update/2
  Weighted slopes/1 -> h over 6/1
  Weight k4/1 -> Weighted slopes/4
  Weight k3/1 -> Weighted slopes/3
  Weight k2/1 -> Weighted slopes/2
  Weight k1/1 -> Weighted slopes/1
  k4/1(xdot) -> Weight k4/1
  Stage state 4/1 -> k4/1(x)
  Stage increment 3/1 -> Stage state 4/2
  k3/1(xdot) -> Weight k3/1, Stage increment 3/1
  Stage state 3/1 -> k3/1(x)
  Stage increment 2/1 -> Stage state 3/2
  k2/1(xdot) -> Weight k2/1, Stage increment 2/1
  Stage state 2/1 -> k2/1(x)
  Stage increment 1/1 -> Stage state 2/2
  k1/1(xdot) -> Weight k1/1, Stage increment 1/1
  tau/1 -> k4/2(tau), k3/2(tau), k2/2(tau), k1/2(tau)
  x/1 -> State update/1, Stage state 4/1, Stage state 3/1, Stage state 2/1, k1/1(x)

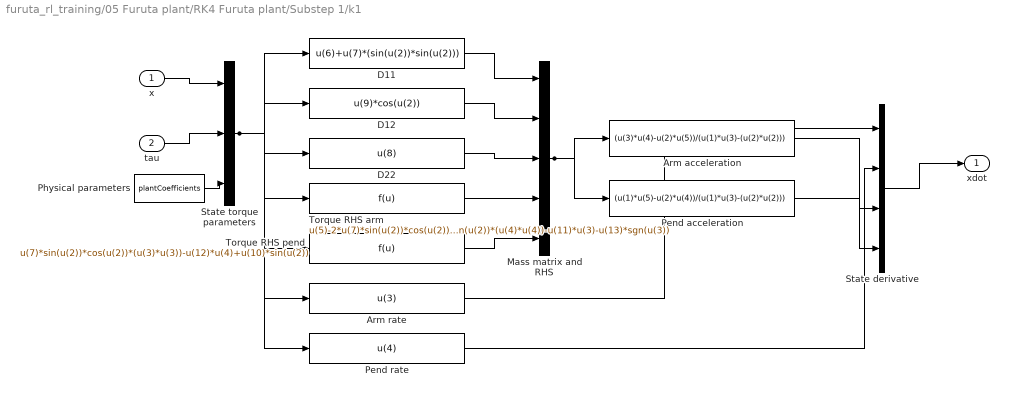
== system furuta_rl_training/05 Furuta plant/RK4 Furuta plant/Substep 1/k1 ==
  x : Inport
  tau : Inport  Port=2
  Arm acceleration : Fcn  Expr=(u(3)*u(4)-u(2)*u(5))/(u(1)*u(3)-(u(2)*u(2)))
  Arm rate : Fcn  Expr=u(3)
  D11 : Fcn  Expr=u(6)+u(7)*(sin(u(2))*sin(u(2)))
  D12 : Fcn  Expr=u(9)*cos(u(2))
  D22 : Fcn  Expr=u(8)
  Mass matrix and RHS : Mux  Inputs=5
  Pend acceleration : Fcn  Expr=(u(1)*u(5)-u(2)*u(4))/(u(1)*u(3)-(u(2)*u(2)))
  Pend rate : Fcn  Expr=u(4)
  Physical parameters : Constant  Value=plantCoefficients
  State derivative : Mux
  State torque parameters : Mux  Inputs=3
  Torque RHS arm : Fcn  Expr=u(5)-2*u(7)*sin(u(2))*cos(u(2))*u(3)*u(4)+u(9)*sin(u(2))*(u(4)*u(4))-u(11)*u(3)-u(13)*sgn(u(3))
  Torque RHS pend : Fcn  Expr=u(7)*sin(u(2))*cos(u(2))*(u(3)*u(3))-u(12)*u(4)+u(10)*sin(u(2))
  xdot : Outport
  wires:
  x/1 -> State torque parameters/1
  tau/1 -> State torque parameters/2
  Physical parameters/1 -> State torque parameters/3
  State torque parameters/1 -> D11/1, D12/1, D22/1, Torque RHS arm/1, Torque RHS pend/1, Arm rate/1, Pend rate/1
  D11/1 -> Mass matrix and RHS/1
  D12/1 -> Mass matrix and RHS/2
  D22/1 -> Mass matrix and RHS/3
  Torque RHS arm/1 -> Mass matrix and RHS/4
  Torque RHS pend/1 -> Mass matrix and RHS/5
  Arm rate/1 -> State derivative/1
  Pend rate/1 -> State derivative/2
  Mass matrix and RHS/1 -> Arm acceleration/1, Pend acceleration/1
  Arm acceleration/1 -> State derivative/3
  Pend acceleration/1 -> State derivative/4
  State derivative/1 -> xdot/1

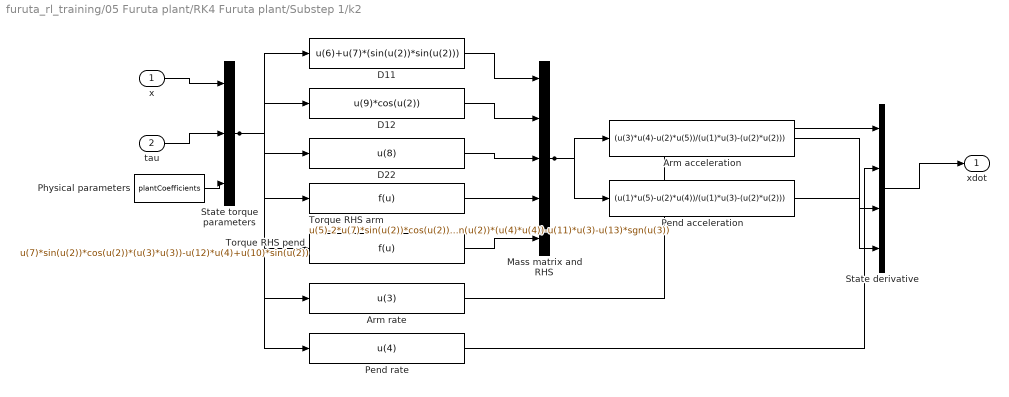
== system furuta_rl_training/05 Furuta plant/RK4 Furuta plant/Substep 1/k2 ==
  x : Inport
  tau : Inport  Port=2
  Arm acceleration : Fcn  Expr=(u(3)*u(4)-u(2)*u(5))/(u(1)*u(3)-(u(2)*u(2)))
  Arm rate : Fcn  Expr=u(3)
  D11 : Fcn  Expr=u(6)+u(7)*(sin(u(2))*sin(u(2)))
  D12 : Fcn  Expr=u(9)*cos(u(2))
  D22 : Fcn  Expr=u(8)
  Mass matrix and RHS : Mux  Inputs=5
  Pend acceleration : Fcn  Expr=(u(1)*u(5)-u(2)*u(4))/(u(1)*u(3)-(u(2)*u(2)))
  Pend rate : Fcn  Expr=u(4)
  Physical parameters : Constant  Value=plantCoefficients
  State derivative : Mux
  State torque parameters : Mux  Inputs=3
  Torque RHS arm : Fcn  Expr=u(5)-2*u(7)*sin(u(2))*cos(u(2))*u(3)*u(4)+u(9)*sin(u(2))*(u(4)*u(4))-u(11)*u(3)-u(13)*sgn(u(3))
  Torque RHS pend : Fcn  Expr=u(7)*sin(u(2))*cos(u(2))*(u(3)*u(3))-u(12)*u(4)+u(10)*sin(u(2))
  xdot : Outport
  wires:
  State derivative/1 -> xdot/1
  Pend acceleration/1 -> State derivative/4
  Arm acceleration/1 -> State derivative/3
  Mass matrix and RHS/1 -> Pend acceleration/1, Arm acceleration/1
  Pend rate/1 -> State derivative/2
  Arm rate/1 -> State derivative/1
  Torque RHS pend/1 -> Mass matrix and RHS/5
  Torque RHS arm/1 -> Mass matrix and RHS/4
  D22/1 -> Mass matrix and RHS/3
  D12/1 -> Mass matrix and RHS/2
  D11/1 -> Mass matrix and RHS/1
  State torque parameters/1 -> Pend rate/1, Arm rate/1, Torque RHS pend/1, Torque RHS arm/1, D22/1, D12/1, D11/1
  Physical parameters/1 -> State torque parameters/3
  tau/1 -> State torque parameters/2
  x/1 -> State torque parameters/1

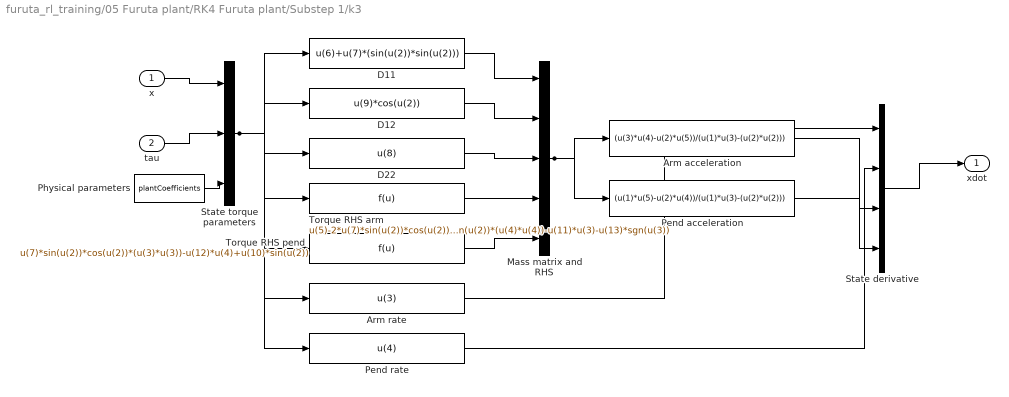
== system furuta_rl_training/05 Furuta plant/RK4 Furuta plant/Substep 1/k3 ==
  x : Inport
  tau : Inport  Port=2
  Arm acceleration : Fcn  Expr=(u(3)*u(4)-u(2)*u(5))/(u(1)*u(3)-(u(2)*u(2)))
  Arm rate : Fcn  Expr=u(3)
  D11 : Fcn  Expr=u(6)+u(7)*(sin(u(2))*sin(u(2)))
  D12 : Fcn  Expr=u(9)*cos(u(2))
  D22 : Fcn  Expr=u(8)
  Mass matrix and RHS : Mux  Inputs=5
  Pend acceleration : Fcn  Expr=(u(1)*u(5)-u(2)*u(4))/(u(1)*u(3)-(u(2)*u(2)))
  Pend rate : Fcn  Expr=u(4)
  Physical parameters : Constant  Value=plantCoefficients
  State derivative : Mux
  State torque parameters : Mux  Inputs=3
  Torque RHS arm : Fcn  Expr=u(5)-2*u(7)*sin(u(2))*cos(u(2))*u(3)*u(4)+u(9)*sin(u(2))*(u(4)*u(4))-u(11)*u(3)-u(13)*sgn(u(3))
  Torque RHS pend : Fcn  Expr=u(7)*sin(u(2))*cos(u(2))*(u(3)*u(3))-u(12)*u(4)+u(10)*sin(u(2))
  xdot : Outport
  wires:
  State derivative/1 -> xdot/1
  Pend acceleration/1 -> State derivative/4
  Arm acceleration/1 -> State derivative/3
  Mass matrix and RHS/1 -> Pend acceleration/1, Arm acceleration/1
  Pend rate/1 -> State derivative/2
  Arm rate/1 -> State derivative/1
  Torque RHS pend/1 -> Mass matrix and RHS/5
  Torque RHS arm/1 -> Mass matrix and RHS/4
  D22/1 -> Mass matrix and RHS/3
  D12/1 -> Mass matrix and RHS/2
  D11/1 -> Mass matrix and RHS/1
  State torque parameters/1 -> Pend rate/1, Arm rate/1, Torque RHS pend/1, Torque RHS arm/1, D22/1, D12/1, D11/1
  Physical parameters/1 -> State torque parameters/3
  tau/1 -> State torque parameters/2
  x/1 -> State torque parameters/1

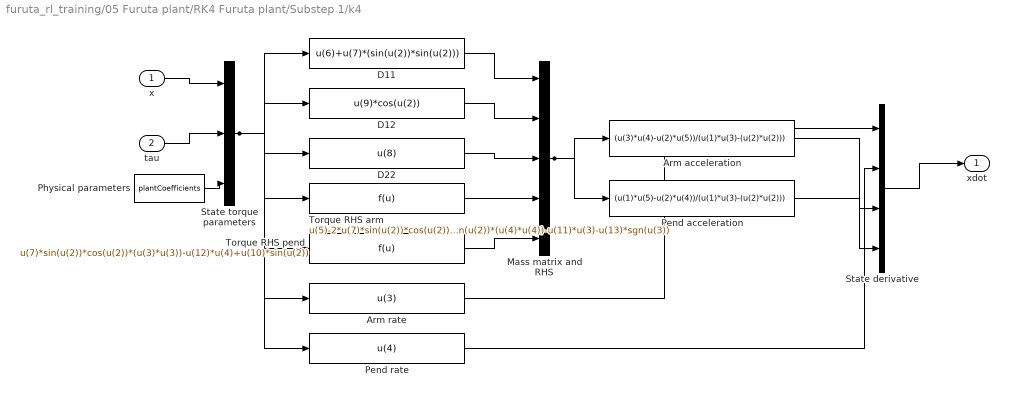
== system furuta_rl_training/05 Furuta plant/RK4 Furuta plant/Substep 1/k4 ==
  x : Inport
  tau : Inport  Port=2
  Arm acceleration : Fcn  Expr=(u(3)*u(4)-u(2)*u(5))/(u(1)*u(3)-(u(2)*u(2)))
  Arm rate : Fcn  Expr=u(3)
  D11 : Fcn  Expr=u(6)+u(7)*(sin(u(2))*sin(u(2)))
  D12 : Fcn  Expr=u(9)*cos(u(2))
  D22 : Fcn  Expr=u(8)
  Mass matrix and RHS : Mux  Inputs=5
  Pend acceleration : Fcn  Expr=(u(1)*u(5)-u(2)*u(4))/(u(1)*u(3)-(u(2)*u(2)))
  Pend rate : Fcn  Expr=u(4)
  Physical parameters : Constant  Value=plantCoefficients
  State derivative : Mux
  State torque parameters : Mux  Inputs=3
  Torque RHS arm : Fcn  Expr=u(5)-2*u(7)*sin(u(2))*cos(u(2))*u(3)*u(4)+u(9)*sin(u(2))*(u(4)*u(4))-u(11)*u(3)-u(13)*sgn(u(3))
  Torque RHS pend : Fcn  Expr=u(7)*sin(u(2))*cos(u(2))*(u(3)*u(3))-u(12)*u(4)+u(10)*sin(u(2))
  xdot : Outport
  wires:
  State derivative/1 -> xdot/1
  Pend acceleration/1 -> State derivative/4
  Arm acceleration/1 -> State derivative/3
  Mass matrix and RHS/1 -> Pend acceleration/1, Arm acceleration/1
  Pend rate/1 -> State derivative/2
  Arm rate/1 -> State derivative/1
  Torque RHS pend/1 -> Mass matrix and RHS/5
  Torque RHS arm/1 -> Mass matrix and RHS/4
  D22/1 -> Mass matrix and RHS/3
  D12/1 -> Mass matrix and RHS/2
  D11/1 -> Mass matrix and RHS/1
  State torque parameters/1 -> Pend rate/1, Arm rate/1, Torque RHS pend/1, Torque RHS arm/1, D22/1, D12/1, D11/1
  Physical parameters/1 -> State torque parameters/3
  tau/1 -> State torque parameters/2
  x/1 -> State torque parameters/1

== system furuta_rl_training/05 Furuta plant/RK4 Furuta plant/Substep 2/k1 ==
  x : Inport
  tau : Inport  Port=2
  Arm acceleration : Fcn  Expr=(u(3)*u(4)-u(2)*u(5))/(u(1)*u(3)-(u(2)*u(2)))
  Arm rate : Fcn  Expr=u(3)
  D11 : Fcn  Expr=u(6)+u(7)*(sin(u(2))*sin(u(2)))
  D12 : Fcn  Expr=u(9)*cos(u(2))
  D22 : Fcn  Expr=u(8)
  Mass matrix and RHS : Mux  Inputs=5
  Pend acceleration : Fcn  Expr=(u(1)*u(5)-u(2)*u(4))/(u(1)*u(3)-(u(2)*u(2)))
  Pend rate : Fcn  Expr=u(4)
  Physical parameters : Constant  Value=plantCoefficients
  State derivative : Mux
  State torque parameters : Mux  Inputs=3
  Torque RHS arm : Fcn  Expr=u(5)-2*u(7)*sin(u(2))*cos(u(2))*u(3)*u(4)+u(9)*sin(u(2))*(u(4)*u(4))-u(11)*u(3)-u(13)*sgn(u(3))
  Torque RHS pend : Fcn  Expr=u(7)*sin(u(2))*cos(u(2))*(u(3)*u(3))-u(12)*u(4)+u(10)*sin(u(2))
  xdot : Outport
  wires:
  State derivative/1 -> xdot/1
  Pend acceleration/1 -> State derivative/4
  Arm acceleration/1 -> State derivative/3
  Mass matrix and RHS/1 -> Pend acceleration/1, Arm acceleration/1
  Pend rate/1 -> State derivative/2
  Arm rate/1 -> State derivative/1
  Torque RHS pend/1 -> Mass matrix and RHS/5
  Torque RHS arm/1 -> Mass matrix and RHS/4
  D22/1 -> Mass matrix and RHS/3
  D12/1 -> Mass matrix and RHS/2
  D11/1 -> Mass matrix and RHS/1
  State torque parameters/1 -> Pend rate/1, Arm rate/1, Torque RHS pend/1, Torque RHS arm/1, D22/1, D12/1, D11/1
  Physical parameters/1 -> State torque parameters/3
  tau/1 -> State torque parameters/2
  x/1 -> State torque parameters/1

== system furuta_rl_training/05 Furuta plant/RK4 Furuta plant/Substep 2/k2 ==
  x : Inport
  tau : Inport  Port=2
  Arm acceleration : Fcn  Expr=(u(3)*u(4)-u(2)*u(5))/(u(1)*u(3)-(u(2)*u(2)))
  Arm rate : Fcn  Expr=u(3)
  D11 : Fcn  Expr=u(6)+u(7)*(sin(u(2))*sin(u(2)))
  D12 : Fcn  Expr=u(9)*cos(u(2))
  D22 : Fcn  Expr=u(8)
  Mass matrix and RHS : Mux  Inputs=5
  Pend acceleration : Fcn  Expr=(u(1)*u(5)-u(2)*u(4))/(u(1)*u(3)-(u(2)*u(2)))
  Pend rate : Fcn  Expr=u(4)
  Physical parameters : Constant  Value=plantCoefficients
  State derivative : Mux
  State torque parameters : Mux  Inputs=3
  Torque RHS arm : Fcn  Expr=u(5)-2*u(7)*sin(u(2))*cos(u(2))*u(3)*u(4)+u(9)*sin(u(2))*(u(4)*u(4))-u(11)*u(3)-u(13)*sgn(u(3))
  Torque RHS pend : Fcn  Expr=u(7)*sin(u(2))*cos(u(2))*(u(3)*u(3))-u(12)*u(4)+u(10)*sin(u(2))
  xdot : Outport
  wires:
  x/1 -> State torque parameters/1
  tau/1 -> State torque parameters/2
  Physical parameters/1 -> State torque parameters/3
  State torque parameters/1 -> D11/1, D12/1, D22/1, Torque RHS arm/1, Torque RHS pend/1, Arm rate/1, Pend rate/1
  D11/1 -> Mass matrix and RHS/1
  D12/1 -> Mass matrix and RHS/2
  D22/1 -> Mass matrix and RHS/3
  Torque RHS arm/1 -> Mass matrix and RHS/4
  Torque RHS pend/1 -> Mass matrix and RHS/5
  Arm rate/1 -> State derivative/1
  Pend rate/1 -> State derivative/2
  Mass matrix and RHS/1 -> Arm acceleration/1, Pend acceleration/1
  Arm acceleration/1 -> State derivative/3
  Pend acceleration/1 -> State derivative/4
  State derivative/1 -> xdot/1

== system furuta_rl_training/05 Furuta plant/RK4 Furuta plant/Substep 2/k3 ==
  x : Inport
  tau : Inport  Port=2
  Arm acceleration : Fcn  Expr=(u(3)*u(4)-u(2)*u(5))/(u(1)*u(3)-(u(2)*u(2)))
  Arm rate : Fcn  Expr=u(3)
  D11 : Fcn  Expr=u(6)+u(7)*(sin(u(2))*sin(u(2)))
  D12 : Fcn  Expr=u(9)*cos(u(2))
  D22 : Fcn  Expr=u(8)
  Mass matrix and RHS : Mux  Inputs=5
  Pend acceleration : Fcn  Expr=(u(1)*u(5)-u(2)*u(4))/(u(1)*u(3)-(u(2)*u(2)))
  Pend rate : Fcn  Expr=u(4)
  Physical parameters : Constant  Value=plantCoefficients
  State derivative : Mux
  State torque parameters : Mux  Inputs=3
  Torque RHS arm : Fcn  Expr=u(5)-2*u(7)*sin(u(2))*cos(u(2))*u(3)*u(4)+u(9)*sin(u(2))*(u(4)*u(4))-u(11)*u(3)-u(13)*sgn(u(3))
  Torque RHS pend : Fcn  Expr=u(7)*sin(u(2))*cos(u(2))*(u(3)*u(3))-u(12)*u(4)+u(10)*sin(u(2))
  xdot : Outport
  wires:
  x/1 -> State torque parameters/1
  tau/1 -> State torque parameters/2
  Physical parameters/1 -> State torque parameters/3
  State torque parameters/1 -> D11/1, D12/1, D22/1, Torque RHS arm/1, Torque RHS pend/1, Arm rate/1, Pend rate/1
  D11/1 -> Mass matrix and RHS/1
  D12/1 -> Mass matrix and RHS/2
  D22/1 -> Mass matrix and RHS/3
  Torque RHS arm/1 -> Mass matrix and RHS/4
  Torque RHS pend/1 -> Mass matrix and RHS/5
  Arm rate/1 -> State derivative/1
  Pend rate/1 -> State derivative/2
  Mass matrix and RHS/1 -> Arm acceleration/1, Pend acceleration/1
  Arm acceleration/1 -> State derivative/3
  Pend acceleration/1 -> State derivative/4
  State derivative/1 -> xdot/1

== system furuta_rl_training/05 Furuta plant/RK4 Furuta plant/Substep 2/k4 ==
  x : Inport
  tau : Inport  Port=2
  Arm acceleration : Fcn  Expr=(u(3)*u(4)-u(2)*u(5))/(u(1)*u(3)-(u(2)*u(2)))
  Arm rate : Fcn  Expr=u(3)
  D11 : Fcn  Expr=u(6)+u(7)*(sin(u(2))*sin(u(2)))
  D12 : Fcn  Expr=u(9)*cos(u(2))
  D22 : Fcn  Expr=u(8)
  Mass matrix and RHS : Mux  Inputs=5
  Pend acceleration : Fcn  Expr=(u(1)*u(5)-u(2)*u(4))/(u(1)*u(3)-(u(2)*u(2)))
  Pend rate : Fcn  Expr=u(4)
  Physical parameters : Constant  Value=plantCoefficients
  State derivative : Mux
  State torque parameters : Mux  Inputs=3
  Torque RHS arm : Fcn  Expr=u(5)-2*u(7)*sin(u(2))*cos(u(2))*u(3)*u(4)+u(9)*sin(u(2))*(u(4)*u(4))-u(11)*u(3)-u(13)*sgn(u(3))
  Torque RHS pend : Fcn  Expr=u(7)*sin(u(2))*cos(u(2))*(u(3)*u(3))-u(12)*u(4)+u(10)*sin(u(2))
  xdot : Outport
  wires:
  x/1 -> State torque parameters/1
  tau/1 -> State torque parameters/2
  Physical parameters/1 -> State torque parameters/3
  State torque parameters/1 -> D11/1, D12/1, D22/1, Torque RHS arm/1, Torque RHS pend/1, Arm rate/1, Pend rate/1
  D11/1 -> Mass matrix and RHS/1
  D12/1 -> Mass matrix and RHS/2
  D22/1 -> Mass matrix and RHS/3
  Torque RHS arm/1 -> Mass matrix and RHS/4
  Torque RHS pend/1 -> Mass matrix and RHS/5
  Arm rate/1 -> State derivative/1
  Pend rate/1 -> State derivative/2
  Mass matrix and RHS/1 -> Arm acceleration/1, Pend acceleration/1
  Arm acceleration/1 -> State derivative/3
  Pend acceleration/1 -> State derivative/4
  State derivative/1 -> xdot/1

== system furuta_rl_training/05 Furuta plant/RK4 Furuta plant/Substep 3/k1 ==
  x : Inport
  tau : Inport  Port=2
  Arm acceleration : Fcn  Expr=(u(3)*u(4)-u(2)*u(5))/(u(1)*u(3)-(u(2)*u(2)))
  Arm rate : Fcn  Expr=u(3)
  D11 : Fcn  Expr=u(6)+u(7)*(sin(u(2))*sin(u(2)))
  D12 : Fcn  Expr=u(9)*cos(u(2))
  D22 : Fcn  Expr=u(8)
  Mass matrix and RHS : Mux  Inputs=5
  Pend acceleration : Fcn  Expr=(u(1)*u(5)-u(2)*u(4))/(u(1)*u(3)-(u(2)*u(2)))
  Pend rate : Fcn  Expr=u(4)
  Physical parameters : Constant  Value=plantCoefficients
  State derivative : Mux
  State torque parameters : Mux  Inputs=3
  Torque RHS arm : Fcn  Expr=u(5)-2*u(7)*sin(u(2))*cos(u(2))*u(3)*u(4)+u(9)*sin(u(2))*(u(4)*u(4))-u(11)*u(3)-u(13)*sgn(u(3))
  Torque RHS pend : Fcn  Expr=u(7)*sin(u(2))*cos(u(2))*(u(3)*u(3))-u(12)*u(4)+u(10)*sin(u(2))
  xdot : Outport
  wires:
  State derivative/1 -> xdot/1
  Pend acceleration/1 -> State derivative/4
  Arm acceleration/1 -> State derivative/3
  Mass matrix and RHS/1 -> Pend acceleration/1, Arm acceleration/1
  Pend rate/1 -> State derivative/2
  Arm rate/1 -> State derivative/1
  Torque RHS pend/1 -> Mass matrix and RHS/5
  Torque RHS arm/1 -> Mass matrix and RHS/4
  D22/1 -> Mass matrix and RHS/3
  D12/1 -> Mass matrix and RHS/2
  D11/1 -> Mass matrix and RHS/1
  State torque parameters/1 -> Pend rate/1, Arm rate/1, Torque RHS pend/1, Torque RHS arm/1, D22/1, D12/1, D11/1
  Physical parameters/1 -> State torque parameters/3
  tau/1 -> State torque parameters/2
  x/1 -> State torque parameters/1

== system furuta_rl_training/05 Furuta plant/RK4 Furuta plant/Substep 3/k2 ==
  x : Inport
  tau : Inport  Port=2
  Arm acceleration : Fcn  Expr=(u(3)*u(4)-u(2)*u(5))/(u(1)*u(3)-(u(2)*u(2)))
  Arm rate : Fcn  Expr=u(3)
  D11 : Fcn  Expr=u(6)+u(7)*(sin(u(2))*sin(u(2)))
  D12 : Fcn  Expr=u(9)*cos(u(2))
  D22 : Fcn  Expr=u(8)
  Mass matrix and RHS : Mux  Inputs=5
  Pend acceleration : Fcn  Expr=(u(1)*u(5)-u(2)*u(4))/(u(1)*u(3)-(u(2)*u(2)))
  Pend rate : Fcn  Expr=u(4)
  Physical parameters : Constant  Value=plantCoefficients
  State derivative : Mux
  State torque parameters : Mux  Inputs=3
  Torque RHS arm : Fcn  Expr=u(5)-2*u(7)*sin(u(2))*cos(u(2))*u(3)*u(4)+u(9)*sin(u(2))*(u(4)*u(4))-u(11)*u(3)-u(13)*sgn(u(3))
  Torque RHS pend : Fcn  Expr=u(7)*sin(u(2))*cos(u(2))*(u(3)*u(3))-u(12)*u(4)+u(10)*sin(u(2))
  xdot : Outport
  wires:
  x/1 -> State torque parameters/1
  tau/1 -> State torque parameters/2
  Physical parameters/1 -> State torque parameters/3
  State torque parameters/1 -> D11/1, D12/1, D22/1, Torque RHS arm/1, Torque RHS pend/1, Arm rate/1, Pend rate/1
  D11/1 -> Mass matrix and RHS/1
  D12/1 -> Mass matrix and RHS/2
  D22/1 -> Mass matrix and RHS/3
  Torque RHS arm/1 -> Mass matrix and RHS/4
  Torque RHS pend/1 -> Mass matrix and RHS/5
  Arm rate/1 -> State derivative/1
  Pend rate/1 -> State derivative/2
  Mass matrix and RHS/1 -> Arm acceleration/1, Pend acceleration/1
  Arm acceleration/1 -> State derivative/3
  Pend acceleration/1 -> State derivative/4
  State derivative/1 -> xdot/1
